simulink model "Bossi_Emanuele_EE460S3D_R99"  (R2025a)
settings: Solver=FixedStepDiscrete  StartTime=0.0  StopTime=120  FixedStep=dt0  RelTol=1e-3  EnableMultiTasking=on
PostLoadFcn:
  | %Set the size for the model
  | set_param(gcs,'Location',[10 10 1270 970])
  | %Set the zoom factor for the model
  | set_param(gcs,'ZoomFactor','100')
InitFcn:
  | tic
  | Bossi_Emanuele_EE460_Final
  | INIT_S3D_01
StartFcn:
  | tend0=toc;
  | tic;
StopFcn:
  | tend=toc;
  | disp(['Simulation time = ' num2str(tout(end)) ' sec'])
  | disp(['Real time = ' num2str(tend) ' sec'])
  | title('DONE')
  | SCORE=round((max(0,120-tout(end)-tend0))*4+10*(40-FuelBurned)+sum(100*double(PDONE)-100*double(PDONE<.5)));
  | PlotS3D(PlotInput);
  | text(15,22,['S: ' num2str(SCORE)]);
  | % Reset color scheme back to normal defaults
  | figure()
  | blkwhitebg('w');
  | close
values from neighbouring files (symbols this model uses):
  A_obs = [ 0  1  0  0  0  0 ... (first row only)    [Bossi_Emanuele_EE460_Final.m]
  B_obs = [ 0     0     0 ... (first row only)    [Bossi_Emanuele_EE460_Final.m]
  C_obs = [ 1 0 0 0 0 0 ... (first row only)    [Bossi_Emanuele_EE460_Final.m]
  d2r = pi/180    (= 0.0174532925199)    [INIT_S3D_01.m]
  D_obs = [ 0     0     0 ... (first row only)    [Bossi_Emanuele_EE460_Final.m]
  dt = 0.01    [INIT_S3D_01.m]
  dt0 = 0.001    [INIT_S3D_01.m]
  fr = 100    [INIT_S3D_01.m]
  G = [1,  1, -1, -1,  0,  0,  0,  0 ... (first row only)    [Bossi_Emanuele_EE460_Final.m]
  G_obs = eye(6)    [Bossi_Emanuele_EE460_Final.m]
  HM_S = 250    [INIT_S3D_01.m]
  HM_U = 500    [INIT_S3D_01.m]
  J = Jbase+JC0+JF+M*(Xcg^2+Ycg^2)    [INIT_S3D_01.m]
  Jbase = JC1+4*Ja+2*Ma*da^2+2*Ma*db^2    [INIT_S3D_01.m]
  JC0 = MC0/2    (= 10.2101761242)    [INIT_S3D_01.m]
  Kdtheta = 2 * zeta_th * wn_th * J_eff    [Bossi_Emanuele_EE460_Final.m]
  Kdtheta_fail = 2 * zeta_th_fail * wn_th_fail * J_eff    [Bossi_Emanuele_EE460_Final.m]
  Kdx = 2 * zeta_xy * wn_xy * M_eff    [Bossi_Emanuele_EE460_Final.m]
  Kdx_fail = 2 * zeta_xy_fail * wn_xy_fail * M_eff    [Bossi_Emanuele_EE460_Final.m]
  Kdy = 2 * zeta_xy * wn_xy * M_eff    [Bossi_Emanuele_EE460_Final.m]
  Kdy_fail = 2 * zeta_xy_fail * wn_xy_fail * M_eff    [Bossi_Emanuele_EE460_Final.m]
  Kptheta = J_eff * wn_th^2    [Bossi_Emanuele_EE460_Final.m]
  Kptheta_fail = J_eff * wn_th_fail^2    [Bossi_Emanuele_EE460_Final.m]
  Kpx = M_eff * wn_xy^2    [Bossi_Emanuele_EE460_Final.m]
  Kpx_fail = M_eff * wn_xy_fail^2    [Bossi_Emanuele_EE460_Final.m]
  Kpy = M_eff * wn_xy^2    [Bossi_Emanuele_EE460_Final.m]
  Kpy_fail = M_eff * wn_xy_fail^2    [Bossi_Emanuele_EE460_Final.m]
  L13 = sqrt(10)    [INIT_S3D_01.m]
  L24 = sqrt(6.25)    [INIT_S3D_01.m]
  LVL = LVL12    [INIT_S3D_01.m]
  M = MC+M1+M2+M3+M4+4*Ma    [INIT_S3D_01.m]
  M1 = LVL.M1    [INIT_S3D_01.m]
  M2 = LVL.M2    [INIT_S3D_01.m]
  M3 = LVL.M3    [INIT_S3D_01.m]
  M4 = LVL.M4    [INIT_S3D_01.m]
  max_qddot = [max_qddot_x; max_qddot_y; max_qddot_theta]    [Bossi_Emanuele_EE460_Final.m]
  mdti = (1/300)    (= 0.00333333333333)    [INIT_S3D_01.m]
  P = [1  1 -1 -1  0  0  0  0 ... (first row only)    [Bossi_Emanuele_EE460_Final.m]
  Pdata = [LVL.P1 LVL.P2 LVL.P3 LVL.P4]    [INIT_S3D_01.m]    (also in PlotS3D.m = R*[xt1;yt1+[0 3*tt*TV(idx-13)*TSIG(idx-13) 0]])
  PTvec = [Pdata(:,1);Pdata(:,2);Pdata(:,3);Pdata(:,4) ... (first row only)    [INIT_S3D_01.m]
  Q_obs = eye(6)    [Bossi_Emanuele_EE460_Final.m]
  r2d = 180/pi    (= 57.2957795131)    [INIT_S3D_01.m]
  r_bang = 0.5    [Bossi_Emanuele_EE460_Final.m]
  Sconfig = 1    [Bossi_Emanuele_EE460_Final.m]
  SLIM = [-100 100 ... (first row only)    [INIT_S3D_01.m]
  SQ = [.005 .01 .004 .005 .01 .004 .02 .01 .4]'    [INIT_S3D_01.m]
  SSF = 1./SQ    [INIT_S3D_01.m]
  tau = 0.5    [Bossi_Emanuele_EE460_Final.m]
  TOLdata = [LVL.P1tol LVL.P2tol LVL.P3tol LVL.P4tol]    [INIT_S3D_01.m]
  ULIM = [[Umin Umax];0 0;0 0]    [INIT_S3D_01.m]
undefined symbols (not defined in the file or in its folder): den_lp, den_lp2, DiscIntNeverNeededParam, dt1_bang_3, dt2_bang_3, dtc_bang_3, num_lp, num_lp2, q0_1
libraries: simulink x87, matrix_library x4, sl3dlib x1, aerolibutil x1, aerolibanimutils x1
(part 4 of 8)

== system Bossi_Emanuele_EE460S3D_R99/ControlLaw/Regulator/NoFailures/AngleWrapper ==
  In1 : Inport
  Atan2 : Trigonometry  Operator=atan2
  Cos : Trigonometry  Operator=cos
  Gain : Gain  Gain=180/pi
  Gain6 : Gain  Gain=pi/180
  Sin : Trigonometry
  Out1 : Outport
  wires:
  Gain6/1 -> Cos/1, Sin/1
  In1/1 -> Gain6/1
  Atan2/1 -> Gain/1
  Gain/1 -> Out1/1  "WrappedAngle_deg"
  Sin/1 -> Atan2/1
  Cos/1 -> Atan2/2

== system Bossi_Emanuele_EE460S3D_R99/ControlLaw/Regulator/ThrusterFailures/AngleWrapper ==
  In1 : Inport
  Atan2 : Trigonometry  Operator=atan2
  Cos : Trigonometry  Operator=cos
  Gain : Gain  Gain=180/pi
  Gain6 : Gain  Gain=pi/180
  Sin : Trigonometry
  Out1 : Outport
  wires:
  Gain6/1 -> Cos/1, Sin/1
  In1/1 -> Gain6/1
  Atan2/1 -> Gain/1
  Gain/1 -> Out1/1  "WrappedAngle_deg"
  Sin/1 -> Atan2/1
  Cos/1 -> Atan2/2

== system Bossi_Emanuele_EE460S3D_R99/S3D_Plant/Comm/P1/DirectionCompensation2 ==
  In1 : Inport
  Compare To Constant : simulink/Logic and Bit Operations/Compare To Constant  relop=<=  const=pi  OutDataTypeStr=boolean
  Compare To Constant1 : simulink/Logic and Bit Operations/Compare To Constant  relop=>=  const=-pi  OutDataTypeStr=boolean
  Constant1 : Constant  Value=2*pi  SampleTime=dt0
  Constant2 : Constant  Value=2*pi  SampleTime=dt0
  Constant3 : Constant  Value=2*pi  SampleTime=dt0
  Mod : Math  Operator=mod
  Sum : Sum  Inputs=|+-
  Sum1 : Sum  Inputs=|++
  Switch : Switch  Criteria=u2 > Threshold  SaturateOnIntegerOverflow=off  InputSameDT=off
  Switch1 : Switch  SaturateOnIntegerOverflow=off  InputSameDT=off
  Switch2 : Switch  Criteria=u2 > Threshold  SaturateOnIntegerOverflow=off  InputSameDT=off
  Out1 : Outport
  wires:
  Sum1/1 -> Switch2/3
  Switch2/1 -> Switch1/3
  Compare To Constant1/1 -> Switch2/2
  Switch/1 -> Switch1/1
  Sum/1 -> Switch/3
  Compare To Constant/1 -> Switch/2
  Mod/1 -> Compare To Constant/1, Sum/1, Switch1/2, Switch2/1, Compare To Constant1/1, Sum1/1, Switch/1
  Switch1/1 -> Out1/1  "Mod_rad"
  Constant2/1 -> Sum1/2
  Constant1/1 -> Sum/2
  In1/1 -> Mod/1
  Constant3/1 -> Mod/2

== system Bossi_Emanuele_EE460S3D_R99/S3D_Plant/Comm/P2/DirectionCompensation2 ==
  In1 : Inport
  Compare To Constant : simulink/Logic and Bit Operations/Compare To Constant  relop=<=  const=pi  OutDataTypeStr=boolean
  Compare To Constant1 : simulink/Logic and Bit Operations/Compare To Constant  relop=>=  const=-pi  OutDataTypeStr=boolean
  Constant1 : Constant  Value=2*pi  SampleTime=dt0
  Constant2 : Constant  Value=2*pi  SampleTime=dt0
  Constant3 : Constant  Value=2*pi  SampleTime=dt0
  Mod : Math  Operator=mod
  Sum : Sum  Inputs=|+-
  Sum1 : Sum  Inputs=|++
  Switch : Switch  Criteria=u2 > Threshold  SaturateOnIntegerOverflow=off  InputSameDT=off
  Switch1 : Switch  SaturateOnIntegerOverflow=off  InputSameDT=off
  Switch2 : Switch  Criteria=u2 > Threshold  SaturateOnIntegerOverflow=off  InputSameDT=off
  Out1 : Outport
  wires:
  Sum1/1 -> Switch2/3
  Switch2/1 -> Switch1/3
  Compare To Constant1/1 -> Switch2/2
  Switch/1 -> Switch1/1
  Sum/1 -> Switch/3
  Compare To Constant/1 -> Switch/2
  Mod/1 -> Compare To Constant/1, Sum/1, Switch1/2, Switch2/1, Compare To Constant1/1, Sum1/1, Switch/1
  Switch1/1 -> Out1/1  "Mod_rad"
  Constant2/1 -> Sum1/2
  Constant1/1 -> Sum/2
  In1/1 -> Mod/1
  Constant3/1 -> Mod/2

== system Bossi_Emanuele_EE460S3D_R99/S3D_Plant/Comm/P3/DirectionCompensation2 ==
  In1 : Inport
  Compare To Constant : simulink/Logic and Bit Operations/Compare To Constant  relop=<=  const=pi  OutDataTypeStr=boolean
  Compare To Constant1 : simulink/Logic and Bit Operations/Compare To Constant  relop=>=  const=-pi  OutDataTypeStr=boolean
  Constant1 : Constant  Value=2*pi  SampleTime=dt0
  Constant2 : Constant  Value=2*pi  SampleTime=dt0
  Constant3 : Constant  Value=2*pi  SampleTime=dt0
  Mod : Math  Operator=mod
  Sum : Sum  Inputs=|+-
  Sum1 : Sum  Inputs=|++
  Switch : Switch  Criteria=u2 > Threshold  SaturateOnIntegerOverflow=off  InputSameDT=off
  Switch1 : Switch  SaturateOnIntegerOverflow=off  InputSameDT=off
  Switch2 : Switch  Criteria=u2 > Threshold  SaturateOnIntegerOverflow=off  InputSameDT=off
  Out1 : Outport
  wires:
  Sum1/1 -> Switch2/3
  Switch2/1 -> Switch1/3
  Compare To Constant1/1 -> Switch2/2
  Switch/1 -> Switch1/1
  Sum/1 -> Switch/3
  Compare To Constant/1 -> Switch/2
  Mod/1 -> Compare To Constant/1, Sum/1, Switch1/2, Switch2/1, Compare To Constant1/1, Sum1/1, Switch/1
  Switch1/1 -> Out1/1  "Mod_rad"
  Constant2/1 -> Sum1/2
  Constant1/1 -> Sum/2
  In1/1 -> Mod/1
  Constant3/1 -> Mod/2

== system Bossi_Emanuele_EE460S3D_R99/S3D_Plant/Comm/P4/DirectionCompensation2 ==
  In1 : Inport
  Compare To Constant : simulink/Logic and Bit Operations/Compare To Constant  relop=<=  const=pi  OutDataTypeStr=boolean
  Compare To Constant1 : simulink/Logic and Bit Operations/Compare To Constant  relop=>=  const=-pi  OutDataTypeStr=boolean
  Constant1 : Constant  Value=2*pi  SampleTime=dt0
  Constant2 : Constant  Value=2*pi  SampleTime=dt0
  Constant3 : Constant  Value=2*pi  SampleTime=dt0
  Mod : Math  Operator=mod
  Sum : Sum  Inputs=|+-
  Sum1 : Sum  Inputs=|++
  Switch : Switch  Criteria=u2 > Threshold  SaturateOnIntegerOverflow=off  InputSameDT=off
  Switch1 : Switch  SaturateOnIntegerOverflow=off  InputSameDT=off
  Switch2 : Switch  Criteria=u2 > Threshold  SaturateOnIntegerOverflow=off  InputSameDT=off
  Out1 : Outport
  wires:
  Sum1/1 -> Switch2/3
  Switch2/1 -> Switch1/3
  Compare To Constant1/1 -> Switch2/2
  Switch/1 -> Switch1/1
  Sum/1 -> Switch/3
  Compare To Constant/1 -> Switch/2
  Mod/1 -> Compare To Constant/1, Sum/1, Switch1/2, Switch2/1, Compare To Constant1/1, Sum1/1, Switch/1
  Switch1/1 -> Out1/1  "Mod_rad"
  Constant2/1 -> Sum1/2
  Constant1/1 -> Sum/2
  In1/1 -> Mod/1
  Constant3/1 -> Mod/2

== system Bossi_Emanuele_EE460S3D_R99/S3D_Plant/Integrate/CentroidData/FindCentroid ==
  MP : Inport
  XCG : Inport  Port=2
  Bus Selector1 : BusSelector  OutputSignals=x_m
  Bus Selector{6..7,9..10} (4 alike) : BusSelector  OutputSignals=tht_rad
  Bus Selector2 : BusSelector  OutputSignals=y_m
  Bus Selector5 : BusSelector  OutputSignals=Xcg_m,Ycg_m
  Bus Selector8 : BusSelector  OutputSignals=Xcg_m,Ycg_m
  Product{2..5} (4 alike) : Product
  Sum1 : Sum  Inputs=|+-
  Sum2 : Sum  Inputs=|+-
  Sum3 : Sum  Inputs=|++
  Sum4 : Sum  Inputs=|+-
  Trigonometric Function2 : Trigonometry
  Trigonometric Function3 : Trigonometry  Operator=cos
  Trigonometric Function4 : Trigonometry  Operator=cos
  Trigonometric Function5 : Trigonometry
  Xcentroid : Outport
  Ycentroid : Outport  Port=2
  wires:
  Bus Selector2/1 -> Sum4/1  "<y_m>"
  Sum2/1 -> Sum1/2
  Bus Selector7/1 -> Trigonometric Function2/1  "<tht_rad>"
  Trigonometric Function4/1 -> Product5/2
  Bus Selector8/2 -> Product5/1  "<Ycg_m>"
  Bus Selector8/1 -> Product4/2  "<Xcg_m>"
  Product5/1 -> Sum3/2
  Bus Selector9/1 -> Trigonometric Function5/1  "<tht_rad>"
  Product4/1 -> Sum3/1
  Bus Selector1/1 -> Sum1/1  "<x_m>"
  Sum1/1 -> Xcentroid/1  "x_m"
  Trigonometric Function3/1 -> Product2/1
  Product3/1 -> Sum2/2
  Bus Selector5/2 -> Product3/1  "<Ycg_m>"
  Bus Selector6/1 -> Trigonometric Function3/1  "<tht_rad>"
  Product2/1 -> Sum2/1
  Bus Selector10/1 -> Trigonometric Function4/1  "<tht_rad>"
  Trigonometric Function5/1 -> Product4/1
  Bus Selector5/1 -> Product2/2  "<Xcg_m>"
  Trigonometric Function2/1 -> Product3/2
  XCG/1 -> Bus Selector10/1, Bus Selector9/1, Bus Selector2/1, Bus Selector7/1, Bus Selector1/1, Bus Selector6/1
  MP/1 -> Bus Selector5/1, Bus Selector8/1
  Sum4/1 -> Ycentroid/1  "y_m"
  Sum3/1 -> Sum4/2

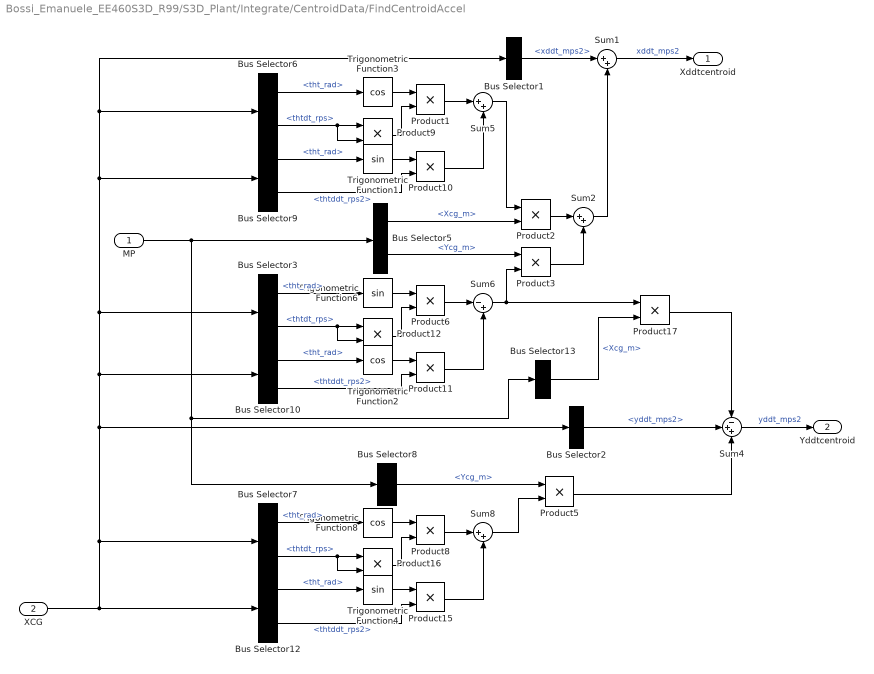
== system Bossi_Emanuele_EE460S3D_R99/S3D_Plant/Integrate/CentroidData/FindCentroidAccel ==
  MP : Inport
  XCG : Inport  Port=2
  Bus Selector1 : BusSelector  OutputSignals=xddt_mps2
  Bus Selector10 : BusSelector  OutputSignals=tht_rad,thtddt_rps2
  Bus Selector12 : BusSelector  OutputSignals=tht_rad,thtddt_rps2
  Bus Selector13 : BusSelector  OutputSignals=Xcg_m
  Bus Selector2 : BusSelector  OutputSignals=yddt_mps2
  Bus Selector3 : BusSelector  OutputSignals=tht_rad,thtdt_rps
  Bus Selector5 : BusSelector  OutputSignals=Xcg_m,Ycg_m
  Bus Selector6 : BusSelector  OutputSignals=tht_rad,thtdt_rps
  Bus Selector7 : BusSelector  OutputSignals=tht_rad,thtdt_rps
  Bus Selector8 : BusSelector  OutputSignals=Ycg_m
  Bus Selector9 : BusSelector  OutputSignals=tht_rad,thtddt_rps2
  Product{1..3,5..6,8..12,15..17} (13 alike) : Product
  Sum{1..2,5,8} (4 alike) : Sum  Inputs=|++
  Sum4 : Sum  Inputs=-++
  Sum6 : Sum  Inputs=|-+
  Trigonometric Function1 : Trigonometry
  Trigonometric Function2 : Trigonometry  Operator=cos
  Trigonometric Function3 : Trigonometry  Operator=cos
  Trigonometric Function4 : Trigonometry
  Trigonometric Function6 : Trigonometry
  Trigonometric Function8 : Trigonometry  Operator=cos
  Xddtcentroid : Outport
  Yddtcentroid : Outport  Port=2
  wires:
  Sum8/1 -> Product5/2
  Product15/1 -> Sum8/2
  Product8/1 -> Sum8/1
  Bus Selector12/2 -> Product15/2  "<thtddt_rps2>"
  Bus Selector12/1 -> Trigonometric Function4/1  "<tht_rad>"
  Trigonometric Function4/1 -> Product15/1
  Product16/1 -> Product8/2
  Bus Selector7/2 -> Product16/1, Product16/2  "<thtdt_rps>"
  Bus Selector7/1 -> Trigonometric Function8/1  "<tht_rad>"
  Trigonometric Function8/1 -> Product8/1
  Sum6/1 -> Product17/1, Product3/2
  Product11/1 -> Sum6/2
  Product6/1 -> Sum6/1
  Bus Selector10/2 -> Product11/2  "<thtddt_rps2>"
  Bus Selector10/1 -> Trigonometric Function2/1  "<tht_rad>"
  Trigonometric Function2/1 -> Product11/1
  Product12/1 -> Product6/2
  Bus Selector3/2 -> Product12/1, Product12/2  "<thtdt_rps>"
  Bus Selector3/1 -> Trigonometric Function6/1  "<tht_rad>"
  Trigonometric Function6/1 -> Product6/1
  Sum5/1 -> Product2/1
  Product10/1 -> Sum5/2
  Product1/1 -> Sum5/1
  Bus Selector9/2 -> Product10/2  "<thtddt_rps2>"
  Bus Selector9/1 -> Trigonometric Function1/1  "<tht_rad>"
  Trigonometric Function1/1 -> Product10/1
  Product9/1 -> Product1/2
  Bus Selector6/2 -> Product9/1, Product9/2  "<thtdt_rps>"
  Bus Selector2/1 -> Sum4/2  "<yddt_mps2>"
  Sum2/1 -> Sum1/2
  Bus Selector1/1 -> Sum1/1  "<xddt_mps2>"
  Sum1/1 -> Xddtcentroid/1  "xddt_mps2"
  Product3/1 -> Sum2/2
  Bus Selector6/1 -> Trigonometric Function3/1  "<tht_rad>"
  Product2/1 -> Sum2/1
  XCG/1 -> Bus Selector12/1, Bus Selector1/1, Bus Selector6/1, Bus Selector9/1, Bus Selector3/1, Bus Selector10/1, Bus Selector2/1, Bus Selector7/1
  MP/1 -> Bus Selector8/1, Bus Selector13/1, Bus Selector5/1
  Sum4/1 -> Yddtcentroid/1  "yddt_mps2"
  Product5/1 -> Sum4/3
  Trigonometric Function3/1 -> Product1/1
  Bus Selector5/1 -> Product2/2  "<Xcg_m>"
  Bus Selector5/2 -> Product3/1  "<Ycg_m>"
  Bus Selector8/1 -> Product5/1  "<Ycg_m>"
  Bus Selector13/1 -> Product17/2  "<Xcg_m>"
  Product17/1 -> Sum4/1

== system Bossi_Emanuele_EE460S3D_R99/S3D_Plant/Integrate/CentroidData/FindCentroidRates ==
  MP : Inport
  XCG : Inport  Port=2
  Bus Selector1 : BusSelector  OutputSignals=xdt_mps
  Bus Selector2 : BusSelector  OutputSignals=ydt_mps
  Bus Selector{3..4,6..7} (4 alike) : BusSelector  OutputSignals=tht_rad,thtdt_rps
  Bus Selector5 : BusSelector  OutputSignals=Xcg_m,Ycg_m
  Bus Selector8 : BusSelector  OutputSignals=Xcg_m,Ycg_m
  Product{1..8} (8 alike) : Product
  Sum1 : Sum  Inputs=|+-
  Sum2 : Sum  Inputs=|--
  Sum3 : Sum  Inputs=|+-
  Sum4 : Sum  Inputs=|+-
  Trigonometric Function2 : Trigonometry  Operator=cos
  Trigonometric Function3 : Trigonometry
  Trigonometric Function4 : Trigonometry
  Trigonometric Function5 : Trigonometry  Operator=cos
  Xdtcentroid : Outport
  Ydtcentroid : Outport  Port=2
  wires:
  Bus Selector7/2 -> Product8/2  "<thtdt_rps>"
  Product8/1 -> Product5/2
  Trigonometric Function4/1 -> Product8/1
  Bus Selector8/2 -> Product5/1  "<Ycg_m>"
  Bus Selector8/1 -> Product4/2  "<Xcg_m>"
  Bus Selector4/2 -> Product7/2  "<thtdt_rps>"
  Product7/1 -> Product4/1
  Trigonometric Function5/1 -> Product7/1
  Product6/1 -> Product3/2
  Bus Selector5/2 -> Product3/1  "<Ycg_m>"
  Bus Selector3/2 -> Product6/2  "<thtdt_rps>"
  Trigonometric Function2/1 -> Product6/1
  Bus Selector5/1 -> Product2/2  "<Xcg_m>"
  Product1/1 -> Product2/1
  Bus Selector6/2 -> Product1/2  "<thtdt_rps>"
  Trigonometric Function3/1 -> Product1/1
  Sum3/1 -> Sum4/2
  Sum4/1 -> Ydtcentroid/1  "ydt_mps"
  MP/1 -> Bus Selector8/1, Bus Selector5/1
  XCG/1 -> Bus Selector3/1, Bus Selector6/1, Bus Selector1/1, Bus Selector2/1, Bus Selector4/1, Bus Selector7/1
  Bus Selector7/1 -> Trigonometric Function4/1  "<tht_rad>"
  Product2/1 -> Sum2/1
  Bus Selector6/1 -> Trigonometric Function3/1  "<tht_rad>"
  Product3/1 -> Sum2/2
  Sum1/1 -> Xdtcentroid/1  "xdt_mps"
  Bus Selector1/1 -> Sum1/1  "<xdt_mps>"
  Product4/1 -> Sum3/1
  Bus Selector4/1 -> Trigonometric Function5/1  "<tht_rad>"
  Product5/1 -> Sum3/2
  Bus Selector3/1 -> Trigonometric Function2/1  "<tht_rad>"
  Sum2/1 -> Sum1/2
  Bus Selector2/1 -> Sum4/1  "<ydt_mps>"

== system Bossi_Emanuele_EE460S3D_R99/S3D_Plant/MassProperties/GetCGnJ/Subsystem ==
  Xmom : Inport
  Ymom : Inport  Port=2
  M_kg : Inport  Port=3
  Product : Product  Inputs=*/
  Product1 : Product  Inputs=*/
  Product2 : Product
  Product3 : Product
  Product4 : Product
  Sum : Sum  Inputs=|++
  Jpat : Outport
  Xcg : Outport  Port=2
  Ycg : Outport  Port=3
  wires:
  Product4/1 -> Jpat/1  "Jpat_kgm2"
  M_kg/1 -> Product/2, Product1/2, Product4/2
  Sum/1 -> Product4/1
  Product3/1 -> Sum/2
  Product2/1 -> Sum/1
  Xmom/1 -> Product/1
  Ymom/1 -> Product1/1
  Product/1 -> Xcg/1, Product2/2, Product2/1  "Xcg_m"
  Product1/1 -> Ycg/1, Product3/1, Product3/2  "Ycg_m"

== system Bossi_Emanuele_EE460S3D_R99/S3D_Plant/OutputDataProcessing/MakePlot/MakePlot ==
  PlotData : Inport
  Interpreted MATLAB Function : MATLABFcn  MATLABFcn=PlotS3D  SampleTime=dt0*fr
  Rate Transition : RateTransition  InitialCondition=[zeros(11,1);0.1*[M1;M2;M3;M4];PTvec;zeros(8,1);0;zeros(8,1);zeros(9,1)]  OutPortSampleTime=dt0*fr
  Terminator : Terminator
  wires:
  PlotData/1 -> Rate Transition/1
  Interpreted MATLAB Function/1 -> Terminator/1
  Rate Transition/1 -> Interpreted MATLAB Function/1

== system Bossi_Emanuele_EE460S3D_R99/S3D_Plant/Sensors/CASE1/THTaccel ==
  X : Inport
  Abs : Abs  SaturateOnIntegerOverflow=off
  Bus Selector3 : BusSelector  OutputSignals=thtddt_rps2
  CURRENT : Subsystem  TreatAsAtomicUnit=on
  Compare To Constant : simulink/Logic and Bit Operations/Compare To Constant  relop=<=  const=0.5  OutDataTypeStr=boolean
  Constant1 : Constant  Value=LVL.Sfail(9)  SampleTime=dt0
  Constant2 : Constant  Value=LVL.Sft(9,1)+rand*(LVL.Sft(9,2)-LVL.Sft(9,1))  SampleTime=dt0
  Digital Clock : DigitalClock  SampleTime=dt0
  Gain : Gain  Gain=LVL.SN
  Gain4 : Gain  Gain=r2d
  If : If  IfExpression=u1 < -0.5  ElseIfExpressions=u1 > 0.5 & u1 < 1.5
  Logical Operator : Logic  Operator=OR  AllPortsSameDT=off  OutDataTypeStr=boolean
  MAX : Subsystem  TreatAsAtomicUnit=on
  MIN : Subsystem  TreatAsAtomicUnit=on
  Merge : Merge  Inputs=3
  Quantizer : Quantizer  QuantizationInterval=SQ(9)  SampleTime=dt0
  Random Number : RandomNumber  Variance=LVL.SigSense(9)  Seed=9  SampleTime=dt0
  Relational Operator : RelationalOperator  Operator=<  OutDataTypeStr=boolean  InputSameDT=off
  Saturation : Saturate  UpperLimit=SLIM(9,2)  LowerLimit=SLIM(9,1)
  Sum : Sum  Inputs=|++
  Switch : Switch  Criteria=u2 > Threshold  SaturateOnIntegerOverflow=off  InputSameDT=off
  Unit Delay : UnitDelay  SampleTime=dt0  HasFrameUpgradeWarning=on
  thtddt1 : Outport
  wires:
  Saturation/1 -> Quantizer/1
  Quantizer/1 -> Unit Delay/1, thtddt1/1
  Gain4/1 -> Sum/1
  Compare To Constant/1 -> Logical Operator/2
  Abs/1 -> Compare To Constant/1
  Constant1/1 -> If/1, Abs/1
  Logical Operator/1 -> Switch/2
  Relational Operator/1 -> Logical Operator/1
  Sum/1 -> Switch/1
  Bus Selector3/1 -> Gain4/1  "<thtddt_rps2>"
  Gain/1 -> Sum/2
  Random Number/1 -> Gain/1
  Merge/1 -> Switch/3
  MIN/1(Out1) -> Merge/1
  CURRENT/1(Out1) -> Merge/3
  X/1 -> Bus Selector3/1
  Constant2/1 -> Relational Operator/2
  MAX/1(Out1) -> Merge/2
  Unit Delay/1 -> CURRENT/1(In1)
  If/3 -> CURRENT/Action
  Digital Clock/1 -> Relational Operator/1
  Switch/1 -> Saturation/1
  If/2 -> MAX/Action
  If/1 -> MIN/Action

== system Bossi_Emanuele_EE460S3D_R99/S3D_Plant/Sensors/CASE1/THTpos1 ==
  X : Inport
  Abs : Abs  SaturateOnIntegerOverflow=off
  Bus Selector3 : BusSelector  OutputSignals=tht_rad
  CURRENT : Subsystem  TreatAsAtomicUnit=on
  Compare To Constant : simulink/Logic and Bit Operations/Compare To Constant  relop=<=  const=0.5  OutDataTypeStr=boolean
  Constant1 : Constant  Value=LVL.Sfail(7)  SampleTime=dt0
  Constant2 : Constant  Value=LVL.Sft(7,1)+rand*(LVL.Sft(7,2)-LVL.Sft(7,1))  SampleTime=dt0
  Digital Clock : DigitalClock  SampleTime=dt0
  Gain : Gain  Gain=LVL.SN
  Gain4 : Gain  Gain=r2d
  If : If  IfExpression=u1 < -0.5  ElseIfExpressions=u1 > 0.5 & u1 < 1.5
  Logical Operator : Logic  Operator=OR  AllPortsSameDT=off  OutDataTypeStr=boolean
  MAX : Subsystem  TreatAsAtomicUnit=on
  MIN : Subsystem  TreatAsAtomicUnit=on
  Merge : Merge  Inputs=3
  Quantizer : Quantizer  QuantizationInterval=SQ(7)  SampleTime=dt0
  Random Number : RandomNumber  Variance=LVL.SigSense(7)  Seed=7  SampleTime=dt0
  Relational Operator : RelationalOperator  Operator=<  OutDataTypeStr=boolean  InputSameDT=off
  Saturation : Saturate  UpperLimit=SLIM(7,2)  LowerLimit=SLIM(7,1)
  Sum : Sum  Inputs=|++
  Switch : Switch  Criteria=u2 > Threshold  SaturateOnIntegerOverflow=off  InputSameDT=off
  Unit Delay : UnitDelay  SampleTime=dt0  HasFrameUpgradeWarning=on
  tht1 : Outport
  wires:
  Saturation/1 -> Quantizer/1
  Switch/1 -> Saturation/1
  Quantizer/1 -> tht1/1, Unit Delay/1
  Gain4/1 -> Sum/1
  Compare To Constant/1 -> Logical Operator/2
  Abs/1 -> Compare To Constant/1
  Constant1/1 -> If/1, Abs/1
  Logical Operator/1 -> Switch/2
  Relational Operator/1 -> Logical Operator/1
  Sum/1 -> Switch/1
  Bus Selector3/1 -> Gain4/1  "<tht_rad>"
  Gain/1 -> Sum/2
  Random Number/1 -> Gain/1
  Merge/1 -> Switch/3
  MIN/1(Out1) -> Merge/1
  CURRENT/1(Out1) -> Merge/3
  X/1 -> Bus Selector3/1
  Constant2/1 -> Relational Operator/2
  MAX/1(Out1) -> Merge/2
  Unit Delay/1 -> CURRENT/1(In1)
  If/3 -> CURRENT/Action
  Digital Clock/1 -> Relational Operator/1
  If/2 -> MAX/Action
  If/1 -> MIN/Action

== system Bossi_Emanuele_EE460S3D_R99/S3D_Plant/Sensors/CASE1/THTvel ==
  X : Inport
  Abs : Abs  SaturateOnIntegerOverflow=off
  Bus Selector3 : BusSelector  OutputSignals=thtdt_rps
  CURRENT : Subsystem  TreatAsAtomicUnit=on
  Compare To Constant : simulink/Logic and Bit Operations/Compare To Constant  relop=<=  const=0.5  OutDataTypeStr=boolean
  Constant1 : Constant  Value=LVL.Sfail(8)  SampleTime=dt0
  Constant2 : Constant  Value=LVL.Sft(8,1)+rand*(LVL.Sft(8,2)-LVL.Sft(8,1))  SampleTime=dt0
  Digital Clock : DigitalClock  SampleTime=dt0
  Gain : Gain  Gain=LVL.SN
  Gain4 : Gain  Gain=r2d
  If : If  IfExpression=u1 < -0.5  ElseIfExpressions=u1 > 0.5 & u1 < 1.5
  Logical Operator : Logic  Operator=OR  AllPortsSameDT=off  OutDataTypeStr=boolean
  MAX : Subsystem  TreatAsAtomicUnit=on
  MIN : Subsystem  TreatAsAtomicUnit=on
  Merge : Merge  Inputs=3
  Quantizer : Quantizer  QuantizationInterval=SQ(8)  SampleTime=dt0
  Random Number : RandomNumber  Variance=LVL.SigSense(8)  Seed=8  SampleTime=dt0
  Relational Operator : RelationalOperator  Operator=<  OutDataTypeStr=boolean  InputSameDT=off
  Saturation : Saturate  UpperLimit=SLIM(8,2)  LowerLimit=SLIM(8,1)
  Sum : Sum  Inputs=|++
  Switch : Switch  Criteria=u2 > Threshold  SaturateOnIntegerOverflow=off  InputSameDT=off
  Unit Delay : UnitDelay  SampleTime=dt0  HasFrameUpgradeWarning=on
  thtdt1 : Outport
  wires:
  Saturation/1 -> Quantizer/1
  Quantizer/1 -> thtdt1/1, Unit Delay/1
  Gain4/1 -> Sum/1
  If/1 -> MIN/Action
  If/2 -> MAX/Action
  Switch/1 -> Saturation/1
  Digital Clock/1 -> Relational Operator/1
  If/3 -> CURRENT/Action
  Unit Delay/1 -> CURRENT/1(In1)
  MAX/1(Out1) -> Merge/2
  Constant2/1 -> Relational Operator/2
  X/1 -> Bus Selector3/1
  CURRENT/1(Out1) -> Merge/3
  MIN/1(Out1) -> Merge/1
  Merge/1 -> Switch/3
  Random Number/1 -> Gain/1
  Gain/1 -> Sum/2
  Bus Selector3/1 -> Gain4/1  "<thtdt_rps>"
  Sum/1 -> Switch/1
  Relational Operator/1 -> Logical Operator/1
  Logical Operator/1 -> Switch/2
  Constant1/1 -> Abs/1, If/1
  Abs/1 -> Compare To Constant/1
  Compare To Constant/1 -> Logical Operator/2

== system Bossi_Emanuele_EE460S3D_R99/S3D_Plant/Sensors/CASE1/Xaccel ==
  X : Inport
  Abs : Abs  SaturateOnIntegerOverflow=off
  Bus Selector3 : BusSelector  OutputSignals=xddt_mps2
  CURRENT : Subsystem  TreatAsAtomicUnit=on
  Compare To Constant : simulink/Logic and Bit Operations/Compare To Constant  relop=<=  const=0.5  OutDataTypeStr=boolean
  Constant1 : Constant  Value=LVL.Sfail(3)  SampleTime=dt0
  Constant2 : Constant  Value=LVL.Sft(3,1)+rand*(LVL.Sft(3,2)-LVL.Sft(3,1))  SampleTime=dt0
  Digital Clock : DigitalClock  SampleTime=dt0
  Gain : Gain  Gain=LVL.SN
  If : If  IfExpression=u1 < -0.5  ElseIfExpressions=u1 > 0.5 & u1 < 1.5
  Logical Operator : Logic  Operator=OR  AllPortsSameDT=off  OutDataTypeStr=boolean
  MAX : Subsystem  TreatAsAtomicUnit=on
  MIN : Subsystem  TreatAsAtomicUnit=on
  Merge : Merge  Inputs=3
  Quantizer : Quantizer  QuantizationInterval=SQ(3)  SampleTime=dt0
  Random Number : RandomNumber  Variance=LVL.SigSense(3)  Seed=3  SampleTime=dt0
  Relational Operator : RelationalOperator  Operator=<  OutDataTypeStr=boolean  InputSameDT=off
  Saturation : Saturate  UpperLimit=SLIM(3,2)  LowerLimit=SLIM(3,1)
  Sum : Sum  Inputs=|++
  Switch : Switch  Criteria=u2 > Threshold  SaturateOnIntegerOverflow=off  InputSameDT=off
  Unit Delay : UnitDelay  SampleTime=dt0  HasFrameUpgradeWarning=on
  xddt1 : Outport
  wires:
  Saturation/1 -> Quantizer/1
  Quantizer/1 -> Unit Delay/1, xddt1/1
  Compare To Constant/1 -> Logical Operator/2
  Abs/1 -> Compare To Constant/1
  Constant1/1 -> If/1, Abs/1
  Logical Operator/1 -> Switch/2
  Relational Operator/1 -> Logical Operator/1
  Sum/1 -> Switch/1
  Bus Selector3/1 -> Sum/1  "<xddt_mps2>"
  Gain/1 -> Sum/2
  Random Number/1 -> Gain/1
  Merge/1 -> Switch/3
  MIN/1(Out1) -> Merge/1
  CURRENT/1(Out1) -> Merge/3
  X/1 -> Bus Selector3/1
  Constant2/1 -> Relational Operator/2
  MAX/1(Out1) -> Merge/2
  Unit Delay/1 -> CURRENT/1(In1)
  If/3 -> CURRENT/Action
  Digital Clock/1 -> Relational Operator/1
  Switch/1 -> Saturation/1
  If/2 -> MAX/Action
  If/1 -> MIN/Action

== system Bossi_Emanuele_EE460S3D_R99/S3D_Plant/Sensors/CASE1/Xpos1 ==
  X : Inport
  Abs : Abs  SaturateOnIntegerOverflow=off
  Bus Selector3 : BusSelector  OutputSignals=x_m
  CURRENT : Subsystem  TreatAsAtomicUnit=on
  Compare To Constant : simulink/Logic and Bit Operations/Compare To Constant  relop=<=  const=0.5  OutDataTypeStr=boolean
  Constant1 : Constant  Value=LVL.Sfail(1)  SampleTime=dt0
  Constant2 : Constant  Value=LVL.Sft(1,1)+rand*(LVL.Sft(1,2)-LVL.Sft(1,1))  SampleTime=dt0
  Digital Clock : DigitalClock  SampleTime=dt0
  Gain : Gain  Gain=LVL.SN
  If : If  IfExpression=u1 < -0.5  ElseIfExpressions=u1 > 0.5 & u1 < 1.5
  Logical Operator : Logic  Operator=OR  AllPortsSameDT=off  OutDataTypeStr=boolean
  MAX : Subsystem  TreatAsAtomicUnit=on
  MIN : Subsystem  TreatAsAtomicUnit=on
  Merge : Merge  Inputs=3
  Quantizer : Quantizer  QuantizationInterval=SQ(1)  SampleTime=dt0
  Random Number : RandomNumber  Variance=LVL.SigSense(1)  Seed=1  SampleTime=dt0
  Relational Operator : RelationalOperator  Operator=<  OutDataTypeStr=boolean  InputSameDT=off
  Saturation : Saturate  UpperLimit=SLIM(1,2)  LowerLimit=SLIM(1,1)
  Sum : Sum  Inputs=|++
  Switch : Switch  Criteria=u2 > Threshold  SaturateOnIntegerOverflow=off  InputSameDT=off
  Unit Delay : UnitDelay  SampleTime=dt0  HasFrameUpgradeWarning=on
  x1 : Outport
  wires:
  Saturation/1 -> Quantizer/1
  Quantizer/1 -> Unit Delay/1, x1/1
  Compare To Constant/1 -> Logical Operator/2
  Abs/1 -> Compare To Constant/1
  Constant1/1 -> If/1, Abs/1
  Logical Operator/1 -> Switch/2
  Relational Operator/1 -> Logical Operator/1
  Sum/1 -> Switch/1
  Bus Selector3/1 -> Sum/1  "<x_m>"
  Gain/1 -> Sum/2
  Random Number/1 -> Gain/1
  Merge/1 -> Switch/3
  MIN/1(Out1) -> Merge/1
  CURRENT/1(Out1) -> Merge/3
  X/1 -> Bus Selector3/1
  Constant2/1 -> Relational Operator/2
  MAX/1(Out1) -> Merge/2
  Unit Delay/1 -> CURRENT/1(In1)
  If/3 -> CURRENT/Action
  Digital Clock/1 -> Relational Operator/1
  Switch/1 -> Saturation/1
  If/2 -> MAX/Action
  If/1 -> MIN/Action

== system Bossi_Emanuele_EE460S3D_R99/S3D_Plant/Sensors/CASE1/Xvel ==
  X : Inport
  Abs : Abs  SaturateOnIntegerOverflow=off
  Bus Selector3 : BusSelector  OutputSignals=xdt_mps
  CURRENT : Subsystem  TreatAsAtomicUnit=on
  Compare To Constant : simulink/Logic and Bit Operations/Compare To Constant  relop=<=  const=0.5  OutDataTypeStr=boolean
  Constant1 : Constant  Value=LVL.Sfail(2)  SampleTime=dt0
  Constant2 : Constant  Value=LVL.Sft(2,1)+rand*(LVL.Sft(2,2)-LVL.Sft(2,1))  SampleTime=dt0
  Digital Clock : DigitalClock  SampleTime=dt0
  Gain : Gain  Gain=LVL.SN
  If : If  IfExpression=u1 < -0.5  ElseIfExpressions=u1 > 0.5 & u1 < 1.5
  Logical Operator : Logic  Operator=OR  AllPortsSameDT=off  OutDataTypeStr=boolean
  MAX : Subsystem  TreatAsAtomicUnit=on
  MIN : Subsystem  TreatAsAtomicUnit=on
  Merge : Merge  Inputs=3
  Quantizer : Quantizer  QuantizationInterval=SQ(2)  SampleTime=dt0
  Random Number : RandomNumber  Variance=LVL.SigSense(2)  Seed=2  SampleTime=dt0
  Relational Operator : RelationalOperator  Operator=<  OutDataTypeStr=boolean  InputSameDT=off
  Saturation : Saturate  UpperLimit=SLIM(2,2)  LowerLimit=SLIM(2,1)
  Sum : Sum  Inputs=|++
  Switch : Switch  Criteria=u2 > Threshold  SaturateOnIntegerOverflow=off  InputSameDT=off
  Unit Delay : UnitDelay  SampleTime=dt0  HasFrameUpgradeWarning=on
  xdt1 : Outport
  wires:
  Saturation/1 -> Quantizer/1
  Quantizer/1 -> xdt1/1, Unit Delay/1
  If/1 -> MIN/Action
  If/2 -> MAX/Action
  Switch/1 -> Saturation/1
  Digital Clock/1 -> Relational Operator/1
  If/3 -> CURRENT/Action
  Unit Delay/1 -> CURRENT/1(In1)
  MAX/1(Out1) -> Merge/2
  Constant2/1 -> Relational Operator/2
  X/1 -> Bus Selector3/1
  CURRENT/1(Out1) -> Merge/3
  MIN/1(Out1) -> Merge/1
  Merge/1 -> Switch/3
  Random Number/1 -> Gain/1
  Gain/1 -> Sum/2
  Bus Selector3/1 -> Sum/1  "<xdt_mps>"
  Sum/1 -> Switch/1
  Relational Operator/1 -> Logical Operator/1
  Logical Operator/1 -> Switch/2
  Constant1/1 -> Abs/1, If/1
  Abs/1 -> Compare To Constant/1
  Compare To Constant/1 -> Logical Operator/2

== system Bossi_Emanuele_EE460S3D_R99/S3D_Plant/Sensors/CASE1/Yaccel ==
  X : Inport
  Abs : Abs  SaturateOnIntegerOverflow=off
  Bus Selector3 : BusSelector  OutputSignals=yddt_mps2
  CURRENT : Subsystem  TreatAsAtomicUnit=on
  Compare To Constant : simulink/Logic and Bit Operations/Compare To Constant  relop=<=  const=0.5  OutDataTypeStr=boolean
  Constant1 : Constant  Value=LVL.Sfail(6)  SampleTime=dt0
  Constant2 : Constant  Value=LVL.Sft(6,1)+rand*(LVL.Sft(6,2)-LVL.Sft(6,1))  SampleTime=dt0
  Digital Clock : DigitalClock  SampleTime=dt0
  Gain : Gain  Gain=LVL.SN
  If : If  IfExpression=u1 < -0.5  ElseIfExpressions=u1 > 0.5 & u1 < 1.5
  Logical Operator : Logic  Operator=OR  AllPortsSameDT=off  OutDataTypeStr=boolean
  MAX : Subsystem  TreatAsAtomicUnit=on
  MIN : Subsystem  TreatAsAtomicUnit=on
  Merge : Merge  Inputs=3
  Quantizer : Quantizer  QuantizationInterval=SQ(6)  SampleTime=dt0
  Random Number : RandomNumber  Variance=LVL.SigSense(6)  Seed=6  SampleTime=dt0
  Relational Operator : RelationalOperator  Operator=<  OutDataTypeStr=boolean  InputSameDT=off
  Saturation : Saturate  UpperLimit=SLIM(6,2)  LowerLimit=SLIM(6,1)
  Sum : Sum  Inputs=|++
  Switch : Switch  Criteria=u2 > Threshold  SaturateOnIntegerOverflow=off  InputSameDT=off
  Unit Delay : UnitDelay  SampleTime=dt0  HasFrameUpgradeWarning=on
  yddt1 : Outport
  wires:
  Saturation/1 -> Quantizer/1
  Quantizer/1 -> yddt1/1, Unit Delay/1
  If/1 -> MIN/Action
  If/2 -> MAX/Action
  Switch/1 -> Saturation/1
  Digital Clock/1 -> Relational Operator/1
  If/3 -> CURRENT/Action
  Unit Delay/1 -> CURRENT/1(In1)
  MAX/1(Out1) -> Merge/2
  Constant2/1 -> Relational Operator/2
  X/1 -> Bus Selector3/1
  CURRENT/1(Out1) -> Merge/3
  MIN/1(Out1) -> Merge/1
  Merge/1 -> Switch/3
  Random Number/1 -> Gain/1
  Gain/1 -> Sum/2
  Bus Selector3/1 -> Sum/1  "<yddt_mps2>"
  Sum/1 -> Switch/1
  Relational Operator/1 -> Logical Operator/1
  Logical Operator/1 -> Switch/2
  Constant1/1 -> Abs/1, If/1
  Abs/1 -> Compare To Constant/1
  Compare To Constant/1 -> Logical Operator/2

== system Bossi_Emanuele_EE460S3D_R99/S3D_Plant/Sensors/CASE1/Ypos1 ==
  X : Inport
  Abs : Abs  SaturateOnIntegerOverflow=off
  Bus Selector3 : BusSelector  OutputSignals=y_m
  CURRENT : Subsystem  TreatAsAtomicUnit=on
  Compare To Constant : simulink/Logic and Bit Operations/Compare To Constant  relop=<=  const=0.5  OutDataTypeStr=boolean
  Constant1 : Constant  Value=LVL.Sfail(4)  SampleTime=dt0
  Constant2 : Constant  Value=LVL.Sft(4,1)+rand*(LVL.Sft(4,2)-LVL.Sft(4,1))  SampleTime=dt0
  Digital Clock : DigitalClock  SampleTime=dt0
  Gain : Gain  Gain=LVL.SN
  If : If  IfExpression=u1 < -0.5  ElseIfExpressions=u1 > 0.5 & u1 < 1.5
  Logical Operator : Logic  Operator=OR  AllPortsSameDT=off  OutDataTypeStr=boolean
  MAX : Subsystem  TreatAsAtomicUnit=on
  MIN : Subsystem  TreatAsAtomicUnit=on
  Merge : Merge  Inputs=3
  Quantizer : Quantizer  QuantizationInterval=SQ(4)  SampleTime=dt0
  Random Number : RandomNumber  Variance=LVL.SigSense(4)  Seed=4  SampleTime=dt0
  Relational Operator : RelationalOperator  Operator=<  OutDataTypeStr=boolean  InputSameDT=off
  Saturation : Saturate  UpperLimit=SLIM(4,2)  LowerLimit=SLIM(4,1)
  Sum : Sum  Inputs=|++
  Switch : Switch  Criteria=u2 > Threshold  SaturateOnIntegerOverflow=off  InputSameDT=off
  Unit Delay : UnitDelay  SampleTime=dt0  HasFrameUpgradeWarning=on
  y1 : Outport
  wires:
  Saturation/1 -> Quantizer/1
  Quantizer/1 -> y1/1, Unit Delay/1
  If/1 -> MIN/Action
  If/2 -> MAX/Action
  Switch/1 -> Saturation/1
  Digital Clock/1 -> Relational Operator/1
  If/3 -> CURRENT/Action
  Unit Delay/1 -> CURRENT/1(In1)
  MAX/1(Out1) -> Merge/2
  Constant2/1 -> Relational Operator/2
  X/1 -> Bus Selector3/1
  CURRENT/1(Out1) -> Merge/3
  MIN/1(Out1) -> Merge/1
  Merge/1 -> Switch/3
  Random Number/1 -> Gain/1
  Gain/1 -> Sum/2
  Bus Selector3/1 -> Sum/1  "<y_m>"
  Sum/1 -> Switch/1
  Relational Operator/1 -> Logical Operator/1
  Logical Operator/1 -> Switch/2
  Constant1/1 -> Abs/1, If/1
  Abs/1 -> Compare To Constant/1
  Compare To Constant/1 -> Logical Operator/2

== system Bossi_Emanuele_EE460S3D_R99/S3D_Plant/Sensors/CASE1/Yvel ==
  X : Inport
  Abs : Abs  SaturateOnIntegerOverflow=off
  Bus Selector3 : BusSelector  OutputSignals=ydt_mps
  CURRENT : Subsystem  TreatAsAtomicUnit=on
  Compare To Constant : simulink/Logic and Bit Operations/Compare To Constant  relop=<=  const=0.5  OutDataTypeStr=boolean
  Constant1 : Constant  Value=LVL.Sfail(5)  SampleTime=dt0
  Constant2 : Constant  Value=LVL.Sft(5,1)+rand*(LVL.Sft(5,2)-LVL.Sft(5,1))  SampleTime=dt0
  Digital Clock : DigitalClock  SampleTime=dt0
  Gain : Gain  Gain=LVL.SN
  If : If  IfExpression=u1 < -0.5  ElseIfExpressions=u1 > 0.5 & u1 < 1.5
  Logical Operator : Logic  Operator=OR  AllPortsSameDT=off  OutDataTypeStr=boolean
  MAX : Subsystem  TreatAsAtomicUnit=on
  MIN : Subsystem  TreatAsAtomicUnit=on
  Merge : Merge  Inputs=3
  Quantizer : Quantizer  QuantizationInterval=SQ(5)  SampleTime=dt0
  Random Number : RandomNumber  Variance=LVL.SigSense(5)  Seed=5  SampleTime=dt0
  Relational Operator : RelationalOperator  Operator=<  OutDataTypeStr=boolean  InputSameDT=off
  Saturation : Saturate  UpperLimit=SLIM(5,2)  LowerLimit=SLIM(5,1)
  Sum : Sum  Inputs=|++
  Switch : Switch  Criteria=u2 > Threshold  SaturateOnIntegerOverflow=off  InputSameDT=off
  Unit Delay : UnitDelay  SampleTime=dt0  HasFrameUpgradeWarning=on
  ydt1 : Outport
  wires:
  Saturation/1 -> Quantizer/1
  Quantizer/1 -> Unit Delay/1, ydt1/1
  Compare To Constant/1 -> Logical Operator/2
  Abs/1 -> Compare To Constant/1
  Constant1/1 -> If/1, Abs/1
  Logical Operator/1 -> Switch/2
  Relational Operator/1 -> Logical Operator/1
  Sum/1 -> Switch/1
  Bus Selector3/1 -> Sum/1  "<ydt_mps>"
  Gain/1 -> Sum/2
  Random Number/1 -> Gain/1
  Merge/1 -> Switch/3
  MIN/1(Out1) -> Merge/1
  CURRENT/1(Out1) -> Merge/3
  X/1 -> Bus Selector3/1
  Constant2/1 -> Relational Operator/2
  MAX/1(Out1) -> Merge/2
  Unit Delay/1 -> CURRENT/1(In1)
  If/3 -> CURRENT/Action
  Digital Clock/1 -> Relational Operator/1
  Switch/1 -> Saturation/1
  If/2 -> MAX/Action
  If/1 -> MIN/Action

== system Bossi_Emanuele_EE460S3D_R99/S3D_Plant/Sensors/CASE2/THTpos1 ==
  X : Inport
  Abs : Abs  SaturateOnIntegerOverflow=off
  Bus Selector3 : BusSelector  OutputSignals=tht_rad
  CURRENT : Subsystem  TreatAsAtomicUnit=on
  Compare To Constant : simulink/Logic and Bit Operations/Compare To Constant  relop=<=  const=0.5  OutDataTypeStr=boolean
  Constant1 : Constant  Value=LVL.Sfail(7)  SampleTime=dt0
  Constant2 : Constant  Value=LVL.Sft(7,1)+rand*(LVL.Sft(7,2)-LVL.Sft(7,1))  SampleTime=dt0
  Digital Clock : DigitalClock  SampleTime=dt0
  Gain : Gain  Gain=LVL.SN
  Gain4 : Gain  Gain=r2d
  If : If  IfExpression=u1 < -0.5  ElseIfExpressions=u1 > 0.5 & u1 < 1.5
  Logical Operator : Logic  Operator=OR  AllPortsSameDT=off  OutDataTypeStr=boolean
  MAX : Subsystem  TreatAsAtomicUnit=on
  MIN : Subsystem  TreatAsAtomicUnit=on
  Merge : Merge  Inputs=3
  Quantizer : Quantizer  QuantizationInterval=SQ(7)  SampleTime=dt0
  Random Number : RandomNumber  Variance=LVL.SigSense(7)  Seed=7  SampleTime=dt0
  Relational Operator : RelationalOperator  Operator=<  OutDataTypeStr=boolean  InputSameDT=off
  Saturation : Saturate  UpperLimit=SLIM(7,2)  LowerLimit=SLIM(7,1)
  Sum : Sum  Inputs=|++
  Switch : Switch  Criteria=u2 > Threshold  SaturateOnIntegerOverflow=off  InputSameDT=off
  Unit Delay : UnitDelay  SampleTime=dt0  HasFrameUpgradeWarning=on
  tht1 : Outport
  wires:
  Saturation/1 -> Quantizer/1
  Switch/1 -> Saturation/1
  If/1 -> MIN/Action
  If/2 -> MAX/Action
  Digital Clock/1 -> Relational Operator/1
  If/3 -> CURRENT/Action
  Unit Delay/1 -> CURRENT/1(In1)
  MAX/1(Out1) -> Merge/2
  Constant2/1 -> Relational Operator/2
  X/1 -> Bus Selector3/1
  CURRENT/1(Out1) -> Merge/3
  MIN/1(Out1) -> Merge/1
  Merge/1 -> Switch/3
  Random Number/1 -> Gain/1
  Gain/1 -> Sum/2
  Bus Selector3/1 -> Gain4/1  "<tht_rad>"
  Sum/1 -> Switch/1
  Relational Operator/1 -> Logical Operator/1
  Logical Operator/1 -> Switch/2
  Constant1/1 -> Abs/1, If/1
  Abs/1 -> Compare To Constant/1
  Compare To Constant/1 -> Logical Operator/2
  Gain4/1 -> Sum/1
  Quantizer/1 -> Unit Delay/1, tht1/1

== system Bossi_Emanuele_EE460S3D_R99/S3D_Plant/Sensors/CASE2/THTpos2 ==
  X : Inport
  Abs : Abs  SaturateOnIntegerOverflow=off
  Bus Selector3 : BusSelector  OutputSignals=tht_rad
  CURRENT : Subsystem  TreatAsAtomicUnit=on
  Compare To Constant : simulink/Logic and Bit Operations/Compare To Constant  relop=<=  const=0.5  OutDataTypeStr=boolean
  Constant1 : Constant  Value=LVL.Sfail(8)  SampleTime=dt0
  Constant2 : Constant  Value=LVL.Sft(8,1)+rand*(LVL.Sft(8,2)-LVL.Sft(8,1))  SampleTime=dt0
  Digital Clock : DigitalClock  SampleTime=dt0
  Gain : Gain  Gain=LVL.SN
  Gain4 : Gain  Gain=r2d
  If : If  IfExpression=u1 < -0.5  ElseIfExpressions=u1 > 0.5 & u1 < 1.5
  Logical Operator : Logic  Operator=OR  AllPortsSameDT=off  OutDataTypeStr=boolean
  MAX : Subsystem  TreatAsAtomicUnit=on
  MIN : Subsystem  TreatAsAtomicUnit=on
  Merge : Merge  Inputs=3
  Quantizer : Quantizer  QuantizationInterval=SQ(7)  SampleTime=dt0
  Random Number : RandomNumber  Variance=LVL.SigSense(7)  Seed=8  SampleTime=dt0
  Relational Operator : RelationalOperator  Operator=<  OutDataTypeStr=boolean  InputSameDT=off
  Saturation : Saturate  UpperLimit=SLIM(7,2)  LowerLimit=SLIM(7,1)
  Sum : Sum  Inputs=|++
  Switch : Switch  Criteria=u2 > Threshold  SaturateOnIntegerOverflow=off  InputSameDT=off
  Unit Delay : UnitDelay  SampleTime=dt0  HasFrameUpgradeWarning=on
  tht1 : Outport
  wires:
  Saturation/1 -> Quantizer/1
  Switch/1 -> Saturation/1
  Quantizer/1 -> Unit Delay/1, tht1/1
  Gain4/1 -> Sum/1
  Compare To Constant/1 -> Logical Operator/2
  Abs/1 -> Compare To Constant/1
  Constant1/1 -> If/1, Abs/1
  Logical Operator/1 -> Switch/2
  Relational Operator/1 -> Logical Operator/1
  Sum/1 -> Switch/1
  Bus Selector3/1 -> Gain4/1  "<tht_rad>"
  Gain/1 -> Sum/2
  Random Number/1 -> Gain/1
  Merge/1 -> Switch/3
  MIN/1(Out1) -> Merge/1
  CURRENT/1(Out1) -> Merge/3
  X/1 -> Bus Selector3/1
  Constant2/1 -> Relational Operator/2
  MAX/1(Out1) -> Merge/2
  Unit Delay/1 -> CURRENT/1(In1)
  If/3 -> CURRENT/Action
  Digital Clock/1 -> Relational Operator/1
  If/2 -> MAX/Action
  If/1 -> MIN/Action

== system Bossi_Emanuele_EE460S3D_R99/S3D_Plant/Sensors/CASE2/THTvel ==
  X : Inport
  Abs : Abs  SaturateOnIntegerOverflow=off
  Bus Selector3 : BusSelector  OutputSignals=thtdt_rps
  CURRENT : Subsystem  TreatAsAtomicUnit=on
  Compare To Constant : simulink/Logic and Bit Operations/Compare To Constant  relop=<=  const=0.5  OutDataTypeStr=boolean
  Constant1 : Constant  Value=LVL.Sfail(9)  SampleTime=dt0
  Constant2 : Constant  Value=LVL.Sft(9,1)+rand*(LVL.Sft(9,2)-LVL.Sft(9,1))  SampleTime=dt0
  Digital Clock : DigitalClock  SampleTime=dt0
  Gain : Gain  Gain=LVL.SN
  Gain4 : Gain  Gain=r2d
  If : If  IfExpression=u1 < -0.5  ElseIfExpressions=u1 > 0.5 & u1 < 1.5
  Logical Operator : Logic  Operator=OR  AllPortsSameDT=off  OutDataTypeStr=boolean
  MAX : Subsystem  TreatAsAtomicUnit=on
  MIN : Subsystem  TreatAsAtomicUnit=on
  Merge : Merge  Inputs=3
  Quantizer : Quantizer  QuantizationInterval=SQ(8)  SampleTime=dt0
  Random Number : RandomNumber  Variance=LVL.SigSense(8)  Seed=9  SampleTime=dt0
  Relational Operator : RelationalOperator  Operator=<  OutDataTypeStr=boolean  InputSameDT=off
  Saturation : Saturate  UpperLimit=SLIM(8,2)  LowerLimit=SLIM(8,1)
  Sum : Sum  Inputs=|++
  Switch : Switch  Criteria=u2 > Threshold  SaturateOnIntegerOverflow=off  InputSameDT=off
  Unit Delay : UnitDelay  SampleTime=dt0  HasFrameUpgradeWarning=on
  thtdt1 : Outport
  wires:
  Saturation/1 -> Quantizer/1
  Compare To Constant/1 -> Logical Operator/2
  Abs/1 -> Compare To Constant/1
  Constant1/1 -> If/1, Abs/1
  Logical Operator/1 -> Switch/2
  Relational Operator/1 -> Logical Operator/1
  Sum/1 -> Switch/1
  Bus Selector3/1 -> Gain4/1  "<thtdt_rps>"
  Gain/1 -> Sum/2
  Random Number/1 -> Gain/1
  Merge/1 -> Switch/3
  MIN/1(Out1) -> Merge/1
  CURRENT/1(Out1) -> Merge/3
  X/1 -> Bus Selector3/1
  Constant2/1 -> Relational Operator/2
  MAX/1(Out1) -> Merge/2
  Unit Delay/1 -> CURRENT/1(In1)
  If/3 -> CURRENT/Action
  Digital Clock/1 -> Relational Operator/1
  Switch/1 -> Saturation/1
  If/2 -> MAX/Action
  If/1 -> MIN/Action
  Gain4/1 -> Sum/1
  Quantizer/1 -> Unit Delay/1, thtdt1/1

== system Bossi_Emanuele_EE460S3D_R99/S3D_Plant/Sensors/CASE2/Xpos1 ==
  X : Inport
  Abs : Abs  SaturateOnIntegerOverflow=off
  Bus Selector3 : BusSelector  OutputSignals=x_m
  CURRENT : Subsystem  TreatAsAtomicUnit=on
  Compare To Constant : simulink/Logic and Bit Operations/Compare To Constant  relop=<=  const=0.5  OutDataTypeStr=boolean
  Constant1 : Constant  Value=LVL.Sfail(1)  SampleTime=dt0
  Constant2 : Constant  Value=LVL.Sft(1,1)+rand*(LVL.Sft(1,2)-LVL.Sft(1,1))  SampleTime=dt0
  Digital Clock : DigitalClock  SampleTime=dt0
  Gain : Gain  Gain=LVL.SN
  If : If  IfExpression=u1 < -0.5  ElseIfExpressions=u1 > 0.5 & u1 < 1.5
  Logical Operator : Logic  Operator=OR  AllPortsSameDT=off  OutDataTypeStr=boolean
  MAX : Subsystem  TreatAsAtomicUnit=on
  MIN : Subsystem  TreatAsAtomicUnit=on
  Merge : Merge  Inputs=3
  Quantizer : Quantizer  QuantizationInterval=SQ(1)  SampleTime=dt0
  Random Number : RandomNumber  Variance=LVL.SigSense(1)  Seed=1  SampleTime=dt0
  Relational Operator : RelationalOperator  Operator=<  OutDataTypeStr=boolean  InputSameDT=off
  Saturation : Saturate  UpperLimit=SLIM(1,2)  LowerLimit=SLIM(1,1)
  Sum : Sum  Inputs=|++
  Switch : Switch  Criteria=u2 > Threshold  SaturateOnIntegerOverflow=off  InputSameDT=off
  Unit Delay : UnitDelay  SampleTime=dt0  HasFrameUpgradeWarning=on
  x1 : Outport
  wires:
  Saturation/1 -> Quantizer/1
  If/1 -> MIN/Action
  If/2 -> MAX/Action
  Switch/1 -> Saturation/1
  Digital Clock/1 -> Relational Operator/1
  If/3 -> CURRENT/Action
  Unit Delay/1 -> CURRENT/1(In1)
  MAX/1(Out1) -> Merge/2
  Constant2/1 -> Relational Operator/2
  X/1 -> Bus Selector3/1
  CURRENT/1(Out1) -> Merge/3
  MIN/1(Out1) -> Merge/1
  Merge/1 -> Switch/3
  Random Number/1 -> Gain/1
  Gain/1 -> Sum/2
  Bus Selector3/1 -> Sum/1  "<x_m>"
  Sum/1 -> Switch/1
  Relational Operator/1 -> Logical Operator/1
  Logical Operator/1 -> Switch/2
  Constant1/1 -> Abs/1, If/1
  Abs/1 -> Compare To Constant/1
  Compare To Constant/1 -> Logical Operator/2
  Quantizer/1 -> x1/1, Unit Delay/1

== system Bossi_Emanuele_EE460S3D_R99/S3D_Plant/Sensors/CASE2/Xpos2 ==
  X : Inport
  Abs : Abs  SaturateOnIntegerOverflow=off
  Bus Selector3 : BusSelector  OutputSignals=x_m
  CURRENT : Subsystem  TreatAsAtomicUnit=on
  Compare To Constant : simulink/Logic and Bit Operations/Compare To Constant  relop=<=  const=0.5  OutDataTypeStr=boolean
  Constant1 : Constant  Value=LVL.Sfail(2)  SampleTime=dt0
  Constant2 : Constant  Value=LVL.Sft(2,1)+rand*(LVL.Sft(2,2)-LVL.Sft(2,1))  SampleTime=dt0
  Digital Clock : DigitalClock  SampleTime=dt0
  Gain : Gain  Gain=LVL.SN
  If : If  IfExpression=u1 < -0.5  ElseIfExpressions=u1 > 0.5 & u1 < 1.5
  Logical Operator : Logic  Operator=OR  AllPortsSameDT=off  OutDataTypeStr=boolean
  MAX : Subsystem  TreatAsAtomicUnit=on
  MIN : Subsystem  TreatAsAtomicUnit=on
  Merge : Merge  Inputs=3
  Quantizer : Quantizer  QuantizationInterval=SQ(1)  SampleTime=dt0
  Random Number : RandomNumber  Variance=LVL.SigSense(1)  Seed=2  SampleTime=dt0
  Relational Operator : RelationalOperator  Operator=<  OutDataTypeStr=boolean  InputSameDT=off
  Saturation : Saturate  UpperLimit=SLIM(1,2)  LowerLimit=SLIM(1,1)
  Sum : Sum  Inputs=|++
  Switch : Switch  Criteria=u2 > Threshold  SaturateOnIntegerOverflow=off  InputSameDT=off
  Unit Delay : UnitDelay  SampleTime=dt0  HasFrameUpgradeWarning=on
  x1 : Outport
  wires:
  Saturation/1 -> Quantizer/1
  Quantizer/1 -> Unit Delay/1, x1/1
  Compare To Constant/1 -> Logical Operator/2
  Abs/1 -> Compare To Constant/1
  Constant1/1 -> If/1, Abs/1
  Logical Operator/1 -> Switch/2
  Relational Operator/1 -> Logical Operator/1
  Sum/1 -> Switch/1
  Bus Selector3/1 -> Sum/1  "<x_m>"
  Gain/1 -> Sum/2
  Random Number/1 -> Gain/1
  Merge/1 -> Switch/3
  MIN/1(Out1) -> Merge/1
  CURRENT/1(Out1) -> Merge/3
  X/1 -> Bus Selector3/1
  Constant2/1 -> Relational Operator/2
  MAX/1(Out1) -> Merge/2
  Unit Delay/1 -> CURRENT/1(In1)
  If/3 -> CURRENT/Action
  Digital Clock/1 -> Relational Operator/1
  Switch/1 -> Saturation/1
  If/2 -> MAX/Action
  If/1 -> MIN/Action

== system Bossi_Emanuele_EE460S3D_R99/S3D_Plant/Sensors/CASE2/Xvel ==
  X : Inport
  Abs : Abs  SaturateOnIntegerOverflow=off
  Bus Selector3 : BusSelector  OutputSignals=xdt_mps
  CURRENT : Subsystem  TreatAsAtomicUnit=on
  Compare To Constant : simulink/Logic and Bit Operations/Compare To Constant  relop=<=  const=0.5  OutDataTypeStr=boolean
  Constant1 : Constant  Value=LVL.Sfail(3)  SampleTime=dt0
  Constant2 : Constant  Value=LVL.Sft(3,1)+rand*(LVL.Sft(3,2)-LVL.Sft(3,1))  SampleTime=dt0
  Digital Clock : DigitalClock  SampleTime=dt0
  Gain : Gain  Gain=LVL.SN
  If : If  IfExpression=u1 < -0.5  ElseIfExpressions=u1 > 0.5 & u1 < 1.5
  Logical Operator : Logic  Operator=OR  AllPortsSameDT=off  OutDataTypeStr=boolean
  MAX : Subsystem  TreatAsAtomicUnit=on
  MIN : Subsystem  TreatAsAtomicUnit=on
  Merge : Merge  Inputs=3
  Quantizer : Quantizer  QuantizationInterval=SQ(2)  SampleTime=dt0
  Random Number : RandomNumber  Variance=LVL.SigSense(2)  Seed=3  SampleTime=dt0
  Relational Operator : RelationalOperator  Operator=<  OutDataTypeStr=boolean  InputSameDT=off
  Saturation : Saturate  UpperLimit=SLIM(2,2)  LowerLimit=SLIM(2,1)
  Sum : Sum  Inputs=|++
  Switch : Switch  Criteria=u2 > Threshold  SaturateOnIntegerOverflow=off  InputSameDT=off
  Unit Delay : UnitDelay  SampleTime=dt0  HasFrameUpgradeWarning=on
  xdt1 : Outport
  wires:
  Saturation/1 -> Quantizer/1
  Compare To Constant/1 -> Logical Operator/2
  Abs/1 -> Compare To Constant/1
  Constant1/1 -> If/1, Abs/1
  Logical Operator/1 -> Switch/2
  Relational Operator/1 -> Logical Operator/1
  Sum/1 -> Switch/1
  Bus Selector3/1 -> Sum/1  "<xdt_mps>"
  Gain/1 -> Sum/2
  Random Number/1 -> Gain/1
  Merge/1 -> Switch/3
  MIN/1(Out1) -> Merge/1
  CURRENT/1(Out1) -> Merge/3
  X/1 -> Bus Selector3/1
  Constant2/1 -> Relational Operator/2
  MAX/1(Out1) -> Merge/2
  Unit Delay/1 -> CURRENT/1(In1)
  If/3 -> CURRENT/Action
  Digital Clock/1 -> Relational Operator/1
  Switch/1 -> Saturation/1
  If/2 -> MAX/Action
  If/1 -> MIN/Action
  Quantizer/1 -> Unit Delay/1, xdt1/1
